simulink model "rover"  (R2025b)
settings: Solver=FixedStepAuto  StartTime=0.0  StopTime=10  RelTol=1e-3
undefined symbols (not defined in the file or in its folder): dspblkCoreblockFVToolHelper, gcbh
settings Model: Creator=Mohamed  LastModifiedBy=Mohamed

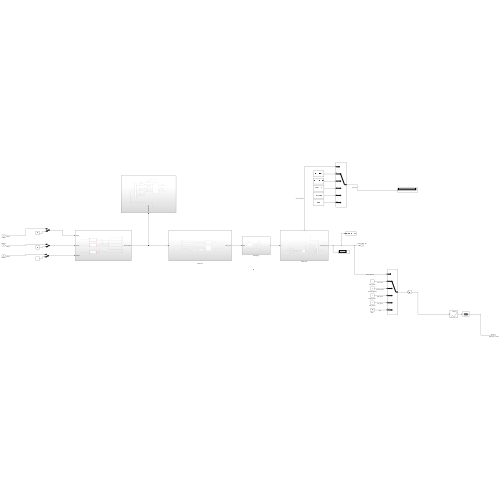
[thumbnail: Simulink's stored preview of the top-level diagram]
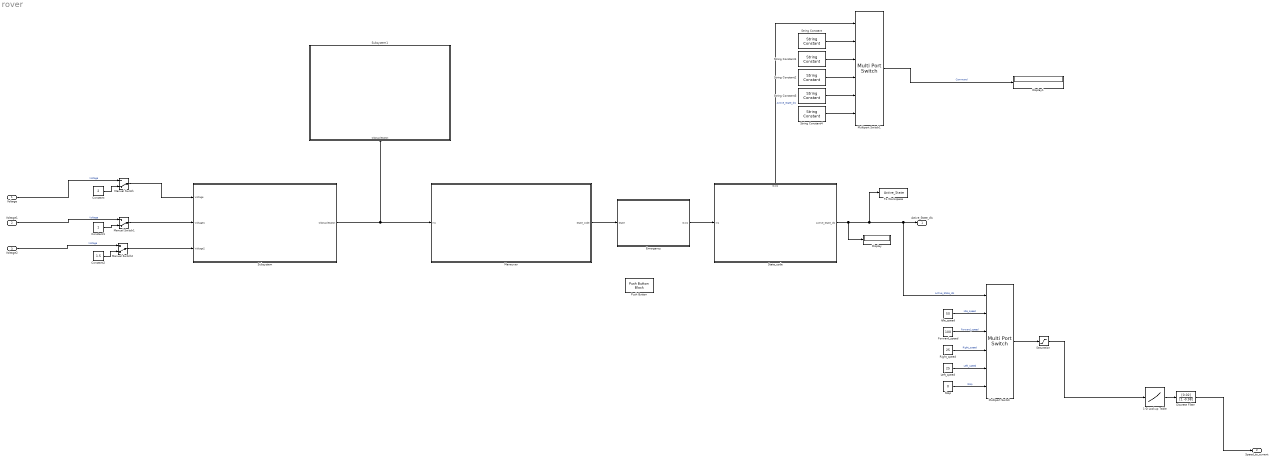
== system rover ==
  Voltage : Inport
  Voltage1 : Inport  Port=2
  Voltage2 : Inport  Port=3
  " Maneuver" : Subsystem
  1-D Lookup Table : Lookup_n-D  NumberOfTableDimensions=1  BreakpointsForDimension1=[0,25,50,100]  Table=[1,15,5,40]  InternalRulePriority=Speed  RndMeth=Simplest
  Constant : Constant  Value=2
  Constant1 : Constant
  Constant2 : Constant  Value=1.5
  Discrete Filter : DiscreteFilter  LoadFcn=dspblkCoreblockFVToolHelper(gcbh,'load');  Numerator=[0.02]  Denominator=[1 -0.98]
      settings: CopyFcn=dspblkCoreblockFVToolHelper(gcbh,'copy');  DeleteFcn=dspblkCoreblockFVToolHelper(gcbh,'close');  ModelCloseFcn=dspblkCoreblockFVToolHelper(gcbh,'close');  PreSaveFcn=dspblkCoreblockFVToolHelper(gcbh,'presave');  PostSaveFcn=dspblkCoreblockFVToolHelper(gcbh,'postsave');  CloseFcn=dspblkCoreblockFVToolHelper(gcbh,'close');
  Display : Display
  Display1 : Display
      settings: Format=long_e
  Emergency : Subsystem
  Forward_speed : Constant  Value=100
  Idle_speed : Constant  Value=50
  Left_speed : Constant  Value=25
  Manual Switch : ManualSwitch  CurrentSetting=0
  Manual Switch1 : ManualSwitch  CurrentSetting=0
  Manual Switch2 : ManualSwitch  CurrentSetting=0
  Multiport Switch : MultiPortSwitch  DataPortOrder=Zero-based contiguous  Inputs=5  zeroidx=on  SaturateOnIntegerOverflow=off  InputSameDT=off
  Multiport Switch1 : MultiPortSwitch  DataPortOrder=Zero-based contiguous  Inputs=5  zeroidx=on  SaturateOnIntegerOverflow=off  InputSameDT=off
  Push Button : PushButtonBlock  IconOnColor=[0.0, 0.39215686274509803, 0.0]  IconOffColor=[0.0, 1.0, 0.0]  OffValue=0.000000
  Right_speed : Constant  Value=25
  Saturation : Saturate  UpperLimit=100  LowerLimit=0
  State_code : Subsystem
      settings: PortSchema="{\"entries\":[{\"content\":{\"sides\":[{\"content\":{\"connectorIds\":[\"In1\"]},\"type\":\"ConnectorPlacement.EquallySpacedRectSide\",\"uuid\":\"04ac484a-7a1a-4432-a070-386b1ef05fea\"},{\"content\":{\"connectorIds\":[\"Out1\"],\"side\":\"RIGHT\"},\"type\":\"ConnectorPlacement.EquallySpacedRectSide\",\"uuid\":\"3dd61b68-c9a6-4f79-b098-a80fc6bac515\"},{\"content\":{\"connectorIds\":[\"Out2\"],\"side\":\"TOP\"},\"type\":\"ConnectorPlacement.EquallySpacedRectSide\",\"uuid\":\"8823efc8-5989-44f2-ab7e-b72cc9bd5ff6\"}]},\"type\":\"ConnectorPlacement.EquallySpacedConnector\",\"uuid\":\"8713e514-aeb9-450c-afe5-19dd3f7905d5\"}],\"packageUris\":[\"http://schema.mathworks.com/mf0/Connector/R2020b\"],\"version\":\"1.0\"}"
  Stop : Constant  Value=0
  String Constant : StringConstant  String="\"IDLE Path\""
  String Constant1 : StringConstant  String="\"FORWARD Path\""
  String Constant2 : StringConstant  String="\"TURN Left\""
  String Constant3 : StringConstant  String="\"TURN Right\""
  String Constant4 : StringConstant  String="\"Stop\""
  Subsystem : Subsystem
  Subsystem1 : Subsystem
      settings: PortSchema="{\"entries\":[{\"content\":{\"sides\":[{\"content\":{},\"type\":\"ConnectorPlacement.EquallySpacedRectSide\",\"uuid\":\"d42d607c-be3e-473f-8fd5-249aa9ef9483\"},{\"content\":{\"side\":\"RIGHT\"},\"type\":\"ConnectorPlacement.EquallySpacedRectSide\",\"uuid\":\"17268d7f-7d5d-4d82-a5c7-3d95164ef75e\"},{\"content\":{\"side\":\"TOP\"},\"type\":\"ConnectorPlacement.EquallySpacedRectSide\",\"uuid\":\"29c6bd7d-c11d-40e8-aad7-06f9da79f2c5\"},{\"content\":{\"connectorIds\":[\"In1\"],\"side\":\"BOTTOM\"},\"type\":\"ConnectorPlacement.EquallySpacedRectSide\",\"uuid\":\"5a0e8200-445f-47b1-872d-66eaa68d9bae\"}]},\"type\":\"ConnectorPlacement.EquallySpacedConnector\",\"uuid\":\"3ecca878-37f1-4558-b5e4-377eafa9f7ec\"}],\"packageUris\":[\"http://schema.mathworks.com/mf0/Connector/R2020b\"],\"version\":\"1.0\"}"
  To Workspace : ToWorkspace  VariableName=Active_State  SaveFormat=Timeseries  SampleTime=-1
  Active_State_dis : Outport
  Speed_to_current : Outport  Port=2
  wires:
  Voltage/1 -> Manual Switch/1  "Voltage"
  Voltage1/1 -> Manual Switch1/1  "Voltage"
  Voltage2/1 -> Manual Switch2/1  "Voltage"
  Subsystem/1(Obstacle&Dist) -> " Maneuver"/1(In1), Subsystem1/1(Obstacle&Dist)
  String Constant3/1 -> Multiport Switch1/5
  String Constant1/1 -> Multiport Switch1/3
  State_code/2(Out1) -> Multiport Switch1/1  "Active_State_dis"
  String Constant2/1 -> Multiport Switch1/4
  String Constant/1 -> Multiport Switch1/2
  Multiport Switch1/1 -> Display1/1  "Command"
  " Maneuver"/1(State_code) -> Emergency/1(State)
  Emergency/1(Out1) -> State_code/1(In1)
  String Constant4/1 -> Multiport Switch1/6
  Manual Switch/1 -> Subsystem/1(Voltage)
  Manual Switch1/1 -> Subsystem/2(Voltage1)
  Manual Switch2/1 -> Subsystem/3(Voltage2)
  Constant/1 -> Manual Switch/2
  Constant1/1 -> Manual Switch1/2
  Constant2/1 -> Manual Switch2/2
  Left_speed/1 -> Multiport Switch/5  "Left_speed"
  State_code/1(Active_State_dis) -> Display/1, To Workspace/1, Multiport Switch/1, Active_State_dis/1  "Active_State_dis"
  Stop/1 -> Multiport Switch/6  "Stop"
  Right_speed/1 -> Multiport Switch/4  "Right_speed"
  Idle_speed/1 -> Multiport Switch/2  "Idle_speed"
  Saturation/1 -> 1-D Lookup Table/1
  Forward_speed/1 -> Multiport Switch/3  "Forward_speed"
  Multiport Switch/1 -> Saturation/1
  1-D Lookup Table/1 -> Discrete Filter/1
  Discrete Filter/1 -> Speed_to_current/1

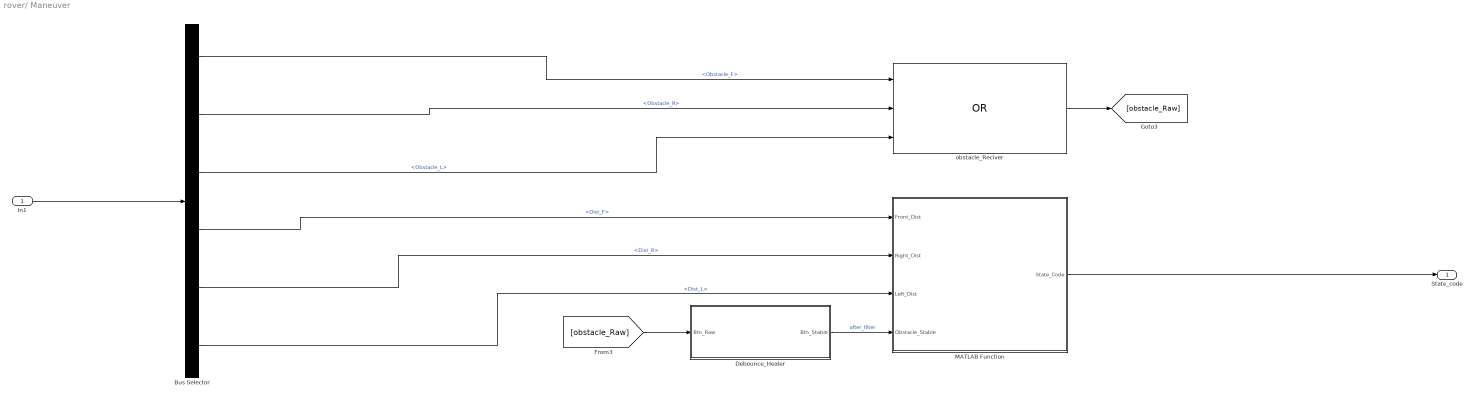
== system rover/ Maneuver ==
  In1 : Inport
  Bus Selector : BusSelector  OutputSignals=Obstacle_F,Obstacle_R,Obstacle_L,Dist_F,Dist_R,Dist_L
  Debounce_Healer : Stateflow chart  TreatAsAtomicUnit=on
  MATLAB Function : MATLAB Function  TreatAsAtomicUnit=on
  obstacle_Reciver : Logic  Operator=OR  Inputs=3  AllPortsSameDT=off  OutDataTypeStr=boolean
  State_code : Outport
  wires:
  Bus Selector/1 -> obstacle_Reciver/1  "<Obstacle_F>"
  Bus Selector/5 -> MATLAB Function/2(Right_Dist)  "<Dist_R>"
  obstacle_Reciver/1 -> [obstacle_Raw]
  Bus Selector/4 -> MATLAB Function/1(Front_Dist)  "<Dist_F>"
  Bus Selector/3 -> obstacle_Reciver/3  "<Obstacle_L>"
  Bus Selector/2 -> obstacle_Reciver/2  "<Obstacle_R>"
  Debounce_Healer/1(Btn_Stable) -> MATLAB Function/4(Obstacle_Stable)  "after_filter"
  Bus Selector/6 -> MATLAB Function/3(Left_Dist)  "<Dist_L>"
  MATLAB Function/1(State_Code) -> State_code/1
  In1/1 -> Bus Selector/1
  [obstacle_Raw] -> Debounce_Healer/1(Btn_Raw)

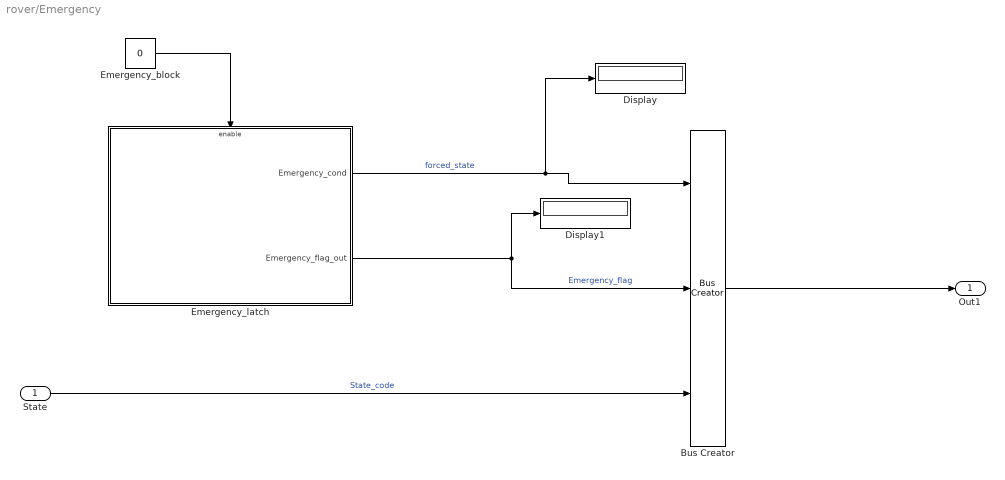
== system rover/Emergency ==
  State : Inport
  Bus Creator : BusCreator  Inputs=3  OutDataTypeStr=Bus: EmergencyStateBus
  Display : Display
  Display1 : Display
  Emergency_block : Constant  Value=0
  Emergency_latch : Subsystem  TreatAsAtomicUnit=on
  Out1 : Outport  OutDataTypeStr=Bus: EmergencyStateBus
  wires:
  Emergency_latch/2(Emergency_flag_out) -> Bus Creator/2, Display1/1  "Emergency_flag"
  Emergency_latch/1(Emergency_cond) -> Display/1, Bus Creator/1  "forced_state"
  State/1 -> Bus Creator/3  "State_code"
  Bus Creator/1 -> Out1/1
  Emergency_block/1 -> Emergency_latch/Enable

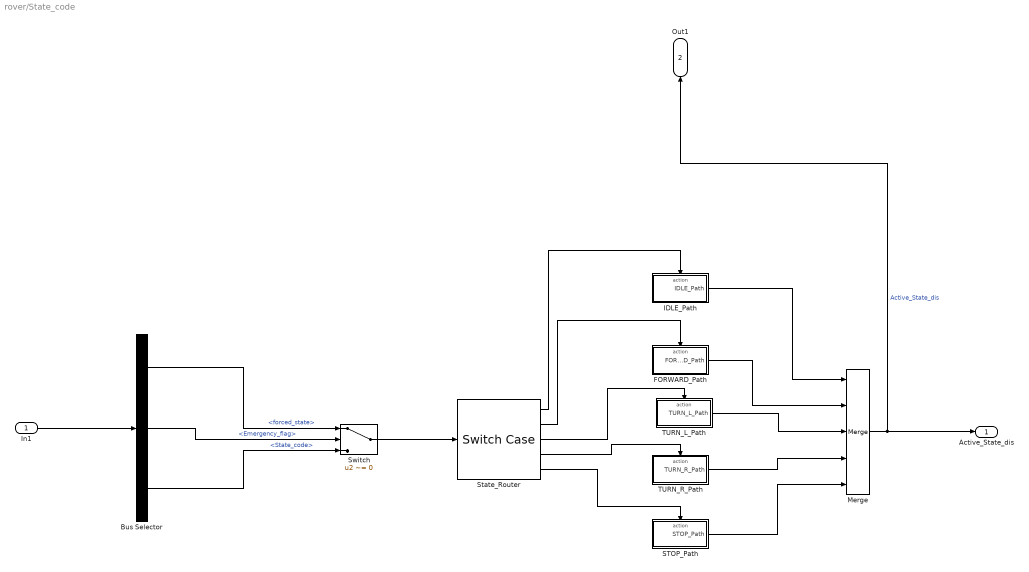
== system rover/State_code ==
  In1 : Inport
  Bus Selector : BusSelector  OutputSignals=forced_state,Emergency_flag,State_code
  FORWARD_Path : Subsystem  TreatAsAtomicUnit=on
  IDLE_Path : Subsystem  TreatAsAtomicUnit=on
  Merge : Merge  Inputs=5
  STOP_Path : Subsystem  TreatAsAtomicUnit=on
  State_Router : SwitchCase  CaseConditions={0,1,2,3,4}  ShowDefaultCase=off
  Switch : Switch  Criteria=u2 ~= 0  SaturateOnIntegerOverflow=off  InputSameDT=off
  TURN_L_Path : Subsystem  TreatAsAtomicUnit=on
  TURN_R_Path : Subsystem  TreatAsAtomicUnit=on
  Active_State_dis : Outport
  Out1 : Outport  Port=2
  wires:
  TURN_R_Path/1(TURN_R_Path) -> Merge/4
  State_Router/4 -> TURN_R_Path/Action
  State_Router/1 -> IDLE_Path/Action
  FORWARD_Path/1(FORWARD_Path) -> Merge/2
  TURN_L_Path/1(TURN_L_Path) -> Merge/3
  STOP_Path/1(STOP_Path) -> Merge/5
  State_Router/2 -> FORWARD_Path/Action
  State_Router/5 -> STOP_Path/Action
  Merge/1 -> Active_State_dis/1, Out1/1  "Active_State_dis"
  IDLE_Path/1(IDLE_Path) -> Merge/1
  State_Router/3 -> TURN_L_Path/Action
  Switch/1 -> State_Router/1
  Bus Selector/3 -> Switch/3  "<State_code>"
  Bus Selector/2 -> Switch/2  "<Emergency_flag>"
  Bus Selector/1 -> Switch/1  "<forced_state>"
  In1/1 -> Bus Selector/1

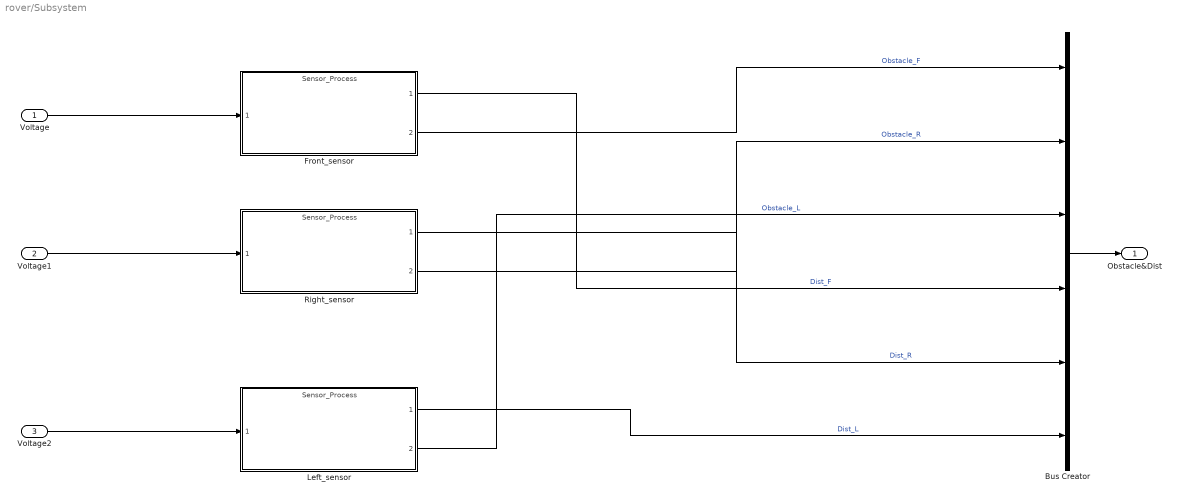
== system rover/Subsystem ==
  Voltage : Inport
  Voltage1 : Inport  Port=2
  Voltage2 : Inport  Port=3
  Bus Creator : BusCreator  Inputs=6  OutDataTypeStr=Bus: SensorArrayBus
  Front_sensor : ModelReference  ModelNameDialog=Sensor_Process.slx  SimulationMode=Normal  ModelReferenceVersion=1.4
  Left_sensor : ModelReference  ModelNameDialog=Sensor_Process.slx  SimulationMode=Normal  ModelReferenceVersion=1.4
  Right_sensor : ModelReference  ModelNameDialog=Sensor_Process.slx  SimulationMode=Normal  ModelReferenceVersion=1.4
  Obstacle&Dist : Outport  OutDataTypeStr=Bus: SensorArrayBus
  wires:
  Voltage2/1 -> Left_sensor/1
  Front_sensor/2 -> Bus Creator/1  "Obstacle_F"
  Voltage1/1 -> Right_sensor/1
  Left_sensor/2 -> Bus Creator/3  "Obstacle_L"
  Left_sensor/1 -> Bus Creator/6  "Dist_L"
  Front_sensor/1 -> Bus Creator/4  "Dist_F"
  Voltage/1 -> Front_sensor/1
  Right_sensor/2 -> Bus Creator/2  "Obstacle_R"
  Right_sensor/1 -> Bus Creator/5  "Dist_R"
  Bus Creator/1 -> Obstacle&Dist/1

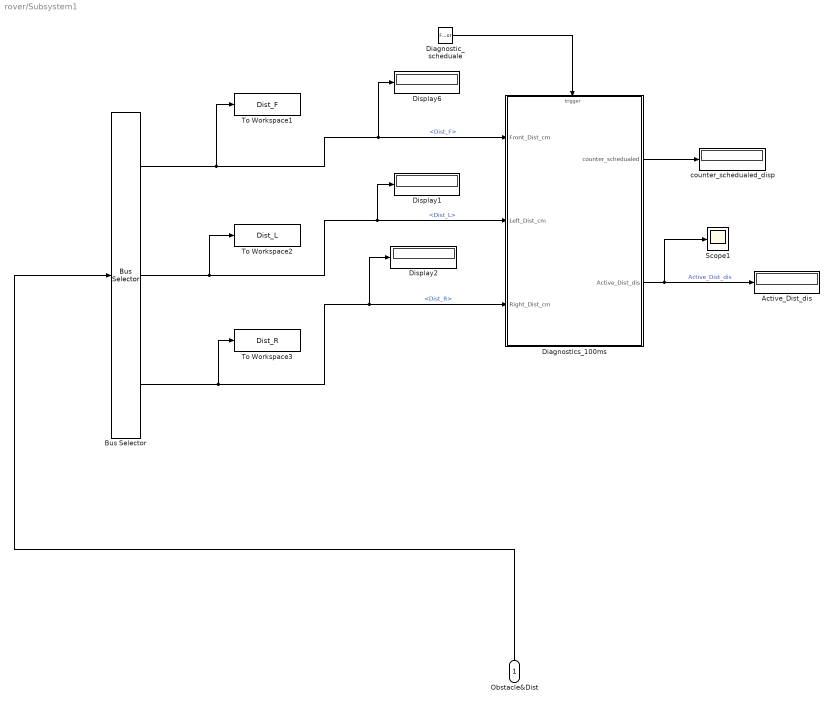
== system rover/Subsystem1 ==
  Obstacle&Dist : Inport
  Active_Dist_dis : Display
  Bus Selector : BusSelector  OutputSignals=Dist_F,Dist_L,Dist_R
  Diagnostic_scheduale : FunctionCallGenerator  SampleTime=0.1
  Diagnostics_100ms : Subsystem  TreatAsAtomicUnit=on
  Display1 : Display
  Display2 : Display
  Display6 : Display
  Scope1 : Scope
      settings: ActiveDisplayYMinimum=-1  ActiveDisplayYMaximum=1
  To Workspace1 : ToWorkspace  VariableName=Dist_F  SaveFormat=Timeseries  SampleTime=-1
  To Workspace2 : ToWorkspace  VariableName=Dist_L  SaveFormat=Timeseries  SampleTime=-1
  To Workspace3 : ToWorkspace  VariableName=Dist_R  SaveFormat=Timeseries  SampleTime=-1
  counter_schedualed_disp : Display
  wires:
  Diagnostics_100ms/1(counter_schedualed) -> counter_schedualed_disp/1
  Diagnostics_100ms/2(Active_Dist_dis) -> Scope1/1, Active_Dist_dis/1  "Active_Dist_dis"
  Diagnostic_scheduale/1 -> Diagnostics_100ms/Trigger
  Obstacle&Dist/1 -> Bus Selector/1
  Bus Selector/1 -> To Workspace1/1, Display6/1, Diagnostics_100ms/1(Front_Dist_cm)  "<Dist_F>"
  Bus Selector/2 -> To Workspace2/1, Display1/1, Diagnostics_100ms/2(Left_Dist_cm)  "<Dist_L>"
  Bus Selector/3 -> To Workspace3/1, Display2/1, Diagnostics_100ms/3(Right_Dist_cm)  "<Dist_R>"

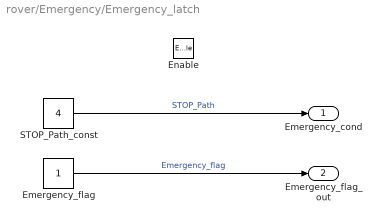
== system rover/Emergency/Emergency_latch ==
  Enable : EnablePort
  Emergency_flag : Constant
  STOP_Path_const : Constant  Value=4
  Emergency_cond : Outport  OutputWhenDisabled=reset  InitialOutput=0
  Emergency_flag_out : Outport  Port=2  OutputWhenDisabled=reset  InitialOutput=0
  wires:
  STOP_Path_const/1 -> Emergency_cond/1  "STOP_Path"
  Emergency_flag/1 -> Emergency_flag_out/1  "Emergency_flag"

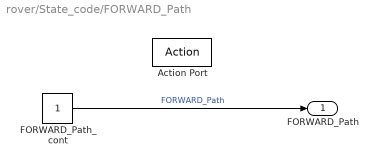
== system rover/State_code/FORWARD_Path ==
  Action Port : ActionPort  ActionPortLabel=case [ 1 ]:
  FORWARD_Path_cont : Constant
  FORWARD_Path : Outport
  wires:
  FORWARD_Path_cont/1 -> FORWARD_Path/1  "FORWARD_Path"

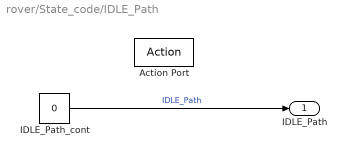
== system rover/State_code/IDLE_Path ==
  Action Port : ActionPort  ActionPortLabel=case [ 0 ]:
  IDLE_Path_cont : Constant  Value=0
  IDLE_Path : Outport
  wires:
  IDLE_Path_cont/1 -> IDLE_Path/1  "IDLE_Path"

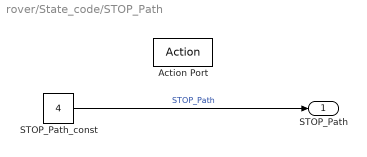
== system rover/State_code/STOP_Path ==
  Action Port : ActionPort  ActionPortLabel=case [ 4 ]:
  STOP_Path_const : Constant  Value=4
  STOP_Path : Outport
  wires:
  STOP_Path_const/1 -> STOP_Path/1  "STOP_Path"

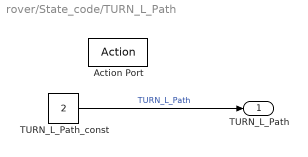
== system rover/State_code/TURN_L_Path ==
  Action Port : ActionPort  ActionPortLabel=case [ 2 ]:
  TURN_L_Path_const : Constant  Value=2
  TURN_L_Path : Outport
  wires:
  TURN_L_Path_const/1 -> TURN_L_Path/1  "TURN_L_Path"

== system rover/State_code/TURN_R_Path ==
  Action Port : ActionPort  ActionPortLabel=case [ 3 ]:
  TURN_R_Path_const : Constant  Value=3
  TURN_R_Path : Outport
  wires:
  TURN_R_Path_const/1 -> TURN_R_Path/1  "TURN_R_Path"

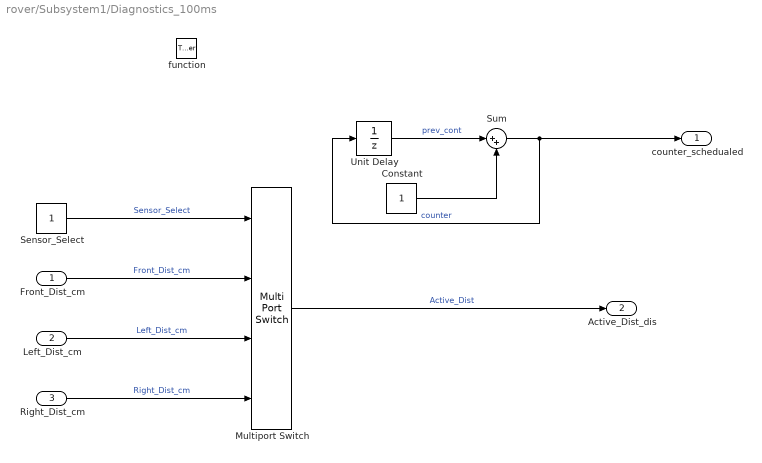
== system rover/Subsystem1/Diagnostics_100ms ==
  Front_Dist_cm : Inport
  Left_Dist_cm : Inport  Port=2
  Right_Dist_cm : Inport  Port=3
  function : TriggerPort  TriggerType=function-call  VariantControl=(inherit)
  Constant : Constant
  Multiport Switch : MultiPortSwitch  SaturateOnIntegerOverflow=off  InputSameDT=off
  Sensor_Select : Constant
  Sum : Sum  Inputs=|++
  Unit Delay : UnitDelay  SampleTime=-1  HasFrameUpgradeWarning=on
  counter_schedualed : Outport
  Active_Dist_dis : Outport  Port=2
  wires:
  Multiport Switch/1 -> Active_Dist_dis/1  "Active_Dist"
  Right_Dist_cm/1 -> Multiport Switch/4  "Right_Dist_cm"
  Front_Dist_cm/1 -> Multiport Switch/2  "Front_Dist_cm"
  Sensor_Select/1 -> Multiport Switch/1  "Sensor_Select"
  Left_Dist_cm/1 -> Multiport Switch/3  "Left_Dist_cm"
  Unit Delay/1 -> Sum/1  "prev_cont"
  Sum/1 -> Unit Delay/1, counter_schedualed/1  "counter"
  Constant/1 -> Sum/2

== matlab function rover/ Maneuver/MATLAB Function ==
  data: Front_Dist input; State_Code output; Right_Dist input; Left_Dist input; Obstacle_Stable input
function State_Code  = DecideRobotState(Front_Dist, Right_Dist, Left_Dist, Obstacle_Stable)

    if Obstacle_Stable && Front_Dist < 20
        State_Code = int32(4);
    elseif Obstacle_Stable && Front_Dist < 40 && Left_Dist > Right_Dist
        State_Code = int32(2);
    elseif Obstacle_Stable && Front_Dist < 40
        State_Code = int32(3);
    elseif Front_Dist >= 40
        State_Code = int32(1);
    else
        State_Code = int32(0);
    end
    
end

== stateflow chart rover/ Maneuver/Debounce_Healer ==
  state ButtonLogic [parallel]
    settings: executionOrder=1
    state Off_Stable
      entry:
      Btn_Stable=0;
      du:
      if(Btn_Raw==false)
      DebounceCounter=0;
      end
    state On_Stable
      entry:
      Btn_Stable=1;
      du:
      if(Btn_Raw==true)
      DebounceCounter=0;
      end
    (junction 31) -> On_Stable [order 2] : [Btn_Raw == 1] /{DebounceCounter = 0;}
    (default) -> Off_Stable
    (junction 31) -> Off_Stable [order 1] : [DebounceCounter >= N_confirm] /{DebounceCounter = 0;}
    On_Stable -> (junction 31) : [Btn_Raw == 0] {DebounceCounter = DebounceCounter + 1;}
    (junction 17) -> On_Stable [order 1] : [DebounceCounter >= N_confirm] /{DebounceCounter = 0;}
    Off_Stable -> (junction 17) : [Btn_Raw == 1] {DebounceCounter = DebounceCounter + 1;}
    (junction 17) -> Off_Stable [order 2] : [Btn_Raw == 0] /{DebounceCounter = 0;}
  (default) -> ButtonLogic
  data: Btn_Raw input boolean; DebounceCounter local int32 =0; N_confirm parameter int32; Btn_Stable output
